simulink model "EV_Bus_Forward_before_readability"  (R2025a)
settings: Solver=ode23t  StartTime=0.0  StopTime=CaseStopTime  MaxStep=Comp.MaxStep  RelTol=1e-5  AbsTol=1e-7
model workspace (MAT data in the model file):
  CaseStopTime = 300
  Comp.Tau = 0.976257419556
  Comp.Limit = 5886
  Comp.InitialForce = 0
  Comp.Enable = 1
  Comp.MinAdaptSpeed = 0.5
  Comp.MeasurementStart = 0
  Comp.MeasurementEnd = 300
  Comp.FilterTau = 0.260335311882
  Comp.Deadband = 44.7421939835
  Comp.ErrorClip = 3531.6
  Comp.MaxRate = 1356.558192
  Comp.LogSampleTime = 0.01
  Comp.MaxStep = 0.01
  MeasuredForceBias = 1114.3044183
  MeasuredTraction = [0 0.01 0.02 0.03 0.04 0.05 0.06 0.07 0.08 0.09 0.1 0.11 ... (60002 elements, 30001x2)]
  P.Mass = 20000
  P.Gravity = 9.81
  P.MotorCount = 2
  P.MotorPower = 400000
  P.MotorPeakTorque = 2500
  P.RegenPeakTorque = 1500
  P.RegenPower = 250000
  P.MaxRPM = 12000
  P.GearRatio = 21
  P.GearEfficiency = 0.97
  P.WheelRadius = 0.5
  P.Cd = 0.65
  P.FrontalArea = 8
  P.Crr = 0.008
  P.AirPressure = 101325
  P.AirGasConstant = 287.05
  P.MotorLag = 0.05
  P.BrakeLag = 0.25
  P.BrakeDelay = 0.1
  P.MaxBrakeTorque = 60000
  P.MaxPressure = 8
  P.DriverKp = 0.22
  P.DriverKi = 0.035
  P.DriverKaw = 2
  P.RegenFadeSpeed = 2
  P.RollingFadeSpeed = 0.2
  P.InitialSpeed = 0
  SignalNames = {'Environment_DesiredSpeed_kmph'; 'Environment_RoadSlope_pct'; 'Environment_AmbientTemp_degC'; 'Driver_Accelerator_pct'; 'Driver_Brake_pct'; 'Powertrain_Controller_MotorCommandTotal_Nm'; 'Powertrain_Controller_BrakeDemandWheel_Nm'; 'Electric_Drive_ActualMotorTotal_Nm'; 'Electric_Drive_ActualMotorEach_Nm'; 'Electric_Drive_ActualMotorSpeed_rpm'; 'Electric_Drive_MechanicalPower_kW'; 'Final_Drive_WheelDriveTorque_Nm'; 'Final_Drive_MotorSpeed_rpm'; 'Final_Drive_FinalDriveRatio'; 'Vehicle_Dynamics_VehicleSpeed_mps'; 'Vehicle_Dynamics_VehicleSpeed_kmph'; 'Vehicle_Dynamics_Acceleration_mps2'; 'Vehicle_Dynamics_AccelerationForce_N'; 'Vehicle_Dynamics_GradientForce_N'; 'Vehicle_Dynamics_RollingResistanceForce_N'; 'Vehicle_Dynamics_AerodynamicForce_N'; 'Vehicle_Dynamics_WheelTractionForce_N'; 'Vehicle_Dynamics_DriveForce_N'; 'Vehicle_Dynamics_FrictionBrakeForce_N'; 'Vehicle_Dynamics_StandstillReaction_N'; 'Vehicle_Dynamics_Distance_m'; 'Pneumatic_Brake_FrictionBrakeTorque_Nm'; 'Pneumatic_Brake_ChamberPressure_bar'; 'MeasuredTraction_N'; 'GenericLossForce_N'; 'CorrectedTraction_N'; 'ResidualError_N'; 'RawDifference_N'; 'AppliedGenericLoss_N'; 'DebiasedMeasuredTraction_N'; 'StationaryForceBias_N'; 'FilteredError_N'; 'AdaptationRate_Nps'}
  SlopeProfile = [0  0; 85  0; 100  4; 140  4; 155  0; 180  -3; 200  0; 300  0]
  SpeedProfile = [0  0; 5  0; 25  40; 55  40; 70  0; 85  0; 105  60; 140  60; 160  40; 180  40; 200  0; 225  0; 245  50; 260  50; 280  0; 300  0]
  TemperatureProfile = [0  25; 150  30; 300  35]
values from neighbouring files (symbols this model uses):
  P =     [EV_Bus_parameters.mat]
(part 1 of 2)
settings Model: Creator=Karuna  LastModifiedBy=Karuna
settings DataIOCC: SignalLogging=off  ReturnWorkspaceOutputs=off

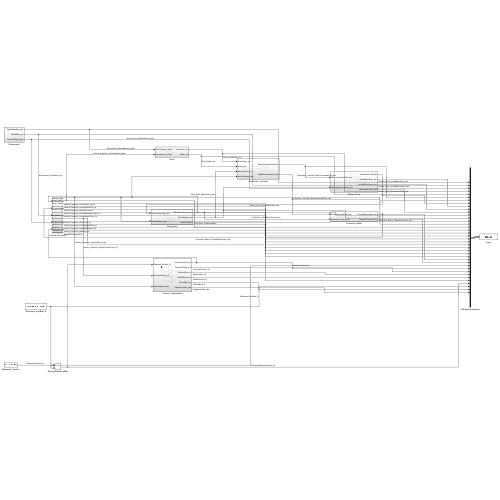
[thumbnail: Simulink's stored preview of the top-level diagram]
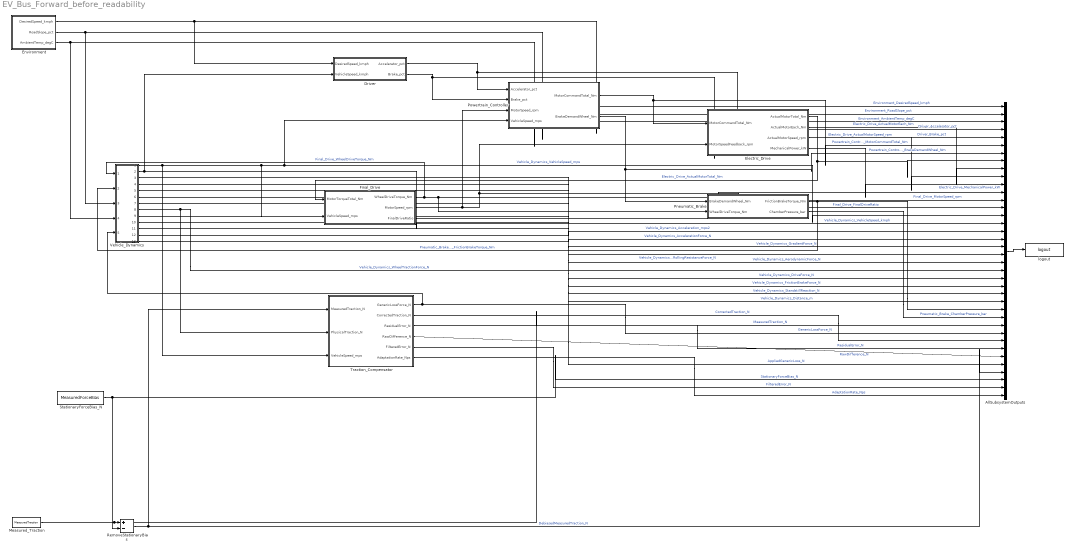
== system EV_Bus_Forward_before_readability ==
  AllSubsystemOutputs : BusCreator  Inputs=38
  Driver : Subsystem  Description=PI speed driver with saturation feedback and integral limits. Non-overlapping accelerator and brake pedals, 0-100%. Minimum 15% holding brake when target <=0.1 km/h.
  Electric_Drive : Subsystem  Description=Equivalent combined model of two identical motors sharing torque equally at common speed. 50 ms torque response; actual torque limited to combined 800 kW drive / 500 kW regen and 5000 / -3000 Nm. Electrical supply assumed available; SOC and thermal dynamics omitted.
  Environment : Subsystem  Description=Linearly interpolated synthetic drive cycle, grade (%) and ambient temperature (degC). Edit SpeedProfile, SlopeProfile and TemperatureProfile in the model workspace.
  Final_Drive : Subsystem  Description=Fixed 21:1 reduction, 0.5 m wheel radius, 97% efficiency. Driving wheel torque = motor torque*21*0.97; regenerative wheel torque = motor torque*21/0.97. RPM comes from actual vehicle speed (no tire slip).
  Measured_Traction : FromWorkspace  Description=MeasuredTraction [relative seconds, signed net traction N], configured by run_EV_Bus_case. Supports arbitrary covered duration and timestamp origin. Original timestamps preserved in logout.sourceTime by the runner.  VariableName=MeasuredTraction
  Pneumatic_Brake : Subsystem  Description=Residual wheel brake demand after actual regenerative torque. Pressure proportional to request, 0.10 s air-line delay and 0.25 s first-order chamber response. 8 bar corresponds to total wheel friction torque 60000 Nm. Reduced-order pneumatic model.
  Powertrain_Controller : Subsystem  Description=Combined command for two equal 400 kW motors. Positive = driving; negative = regeneration. Torque/power envelope, overspeed traction inhibition and regen fade below 2 m/s. Service braking demand is total wheel torque.
  RemoveStationaryBias : Sum  Inputs=+-
  StationaryForceBias_N : Constant  Description=Case-specific measured-force sensor bias. Explicit Bias_N or a user-designated stationary, level, zero-net-traction window; otherwise zero. No universal assumption that the beginning of a recording is stationary.  Value=MeasuredForceBias
  Traction_Compensator : Subsystem  Description=Reusable noise-aware physical loss estimator. All gains, filtering, clipping, bounds and rate limits are in Comp. run_EV_Bus_case imports synchronized measurements/profiles, scales settings from vehicle capability and noise, assesses candidates against a disabled baseline, and checks late-interval performance. Basic Simulink blocks only. Read GENERIC_COMPENSATOR.md for data contract and validity boundaries.
  Vehicle_Dynamics : Subsystem  Description=Physical forward dynamics and traction sum both include AppliedGenericLoss_N. Applied loss = held signed estimate * clamp(v/Comp.MinAdaptSpeed,0,1). Generic motion resistance vanishes at rest; grade is modeled separately. Both force balance identities retained. Ideal standstill constraint can cause abrupt force transitions.
  logout : ToWorkspace  VariableName=logout  SaveFormat=Structure With Time  SampleTime=Comp.LogSampleTime
  wires:
  AllSubsystemOutputs/1 -> logout/1
  Pneumatic_Brake/2(ChamberPressure_bar) -> AllSubsystemOutputs/28  "Pneumatic_Brake_ChamberPressure_bar"
  Final_Drive/3(FinalDriveRatio) -> AllSubsystemOutputs/14  "Final_Drive_FinalDriveRatio"
  Electric_Drive/4(MechanicalPower_kW) -> AllSubsystemOutputs/11  "Electric_Drive_MechanicalPower_kW"
  Electric_Drive/3(ActualMotorSpeed_rpm) -> AllSubsystemOutputs/10  "Electric_Drive_ActualMotorSpeed_rpm"
  Electric_Drive/2(ActualMotorEach_Nm) -> AllSubsystemOutputs/9  "Electric_Drive_ActualMotorEach_Nm"
  Powertrain_Controller/2(BrakeDemandWheel_Nm) -> Pneumatic_Brake/1(BrakeDemandWheel_Nm), AllSubsystemOutputs/7  "Powertrain_Controller_BrakeDemandWheel_Nm"
  Electric_Drive/1(ActualMotorTotal_Nm) -> Final_Drive/1(MotorTorqueTotal_Nm), AllSubsystemOutputs/8  "Electric_Drive_ActualMotorTotal_Nm"
  Powertrain_Controller/1(MotorCommandTotal_Nm) -> Electric_Drive/1(MotorCommandTotal_Nm), AllSubsystemOutputs/6  "Powertrain_Controller_MotorCommandTotal_Nm"
  Final_Drive/2(MotorSpeed_rpm) -> Electric_Drive/2(MotorSpeedFeedback_rpm), AllSubsystemOutputs/13, Powertrain_Controller/3(MotorSpeed_rpm)  "Final_Drive_MotorSpeed_rpm"
  Driver/2(Brake_pct) -> Powertrain_Controller/2(Brake_pct), AllSubsystemOutputs/5  "Driver_Brake_pct"
  Driver/1(Accelerator_pct) -> Powertrain_Controller/1(Accelerator_pct), AllSubsystemOutputs/4  "Driver_Accelerator_pct"
  Environment/1(DesiredSpeed_kmph) -> Driver/1(DesiredSpeed_kmph), AllSubsystemOutputs/1  "Environment_DesiredSpeed_kmph"
  StationaryForceBias_N/1 -> AllSubsystemOutputs/36, RemoveStationaryBias/2  "StationaryForceBias_N"
  Measured_Traction/1 -> RemoveStationaryBias/1, AllSubsystemOutputs/29  "MeasuredTraction_N"
  Vehicle_Dynamics/12(Distance_m) -> AllSubsystemOutputs/26  "Vehicle_Dynamics_Distance_m"
  Vehicle_Dynamics/11(StandstillReaction_N) -> AllSubsystemOutputs/25  "Vehicle_Dynamics_StandstillReaction_N"
  Vehicle_Dynamics/10(FrictionBrakeForce_N) -> AllSubsystemOutputs/24  "Vehicle_Dynamics_FrictionBrakeForce_N"
  Vehicle_Dynamics/9(DriveForce_N) -> AllSubsystemOutputs/23  "Vehicle_Dynamics_DriveForce_N"
  Vehicle_Dynamics/7(AerodynamicForce_N) -> AllSubsystemOutputs/21  "Vehicle_Dynamics_AerodynamicForce_N"
  Vehicle_Dynamics/6(RollingResistanceForce_N) -> AllSubsystemOutputs/20  "Vehicle_Dynamics_RollingResistanceForce_N"
  Vehicle_Dynamics/5(GradientForce_N) -> AllSubsystemOutputs/19  "Vehicle_Dynamics_GradientForce_N"
  Vehicle_Dynamics/4(AccelerationForce_N) -> AllSubsystemOutputs/18  "Vehicle_Dynamics_AccelerationForce_N"
  Vehicle_Dynamics/3(Acceleration_mps2) -> AllSubsystemOutputs/17  "Vehicle_Dynamics_Acceleration_mps2"
  Environment/3(AmbientTemp_degC) -> AllSubsystemOutputs/3, Vehicle_Dynamics/4(AmbientTemp_degC)  "Environment_AmbientTemp_degC"
  Environment/2(RoadSlope_pct) -> Vehicle_Dynamics/3(RoadSlope_pct), AllSubsystemOutputs/2  "Environment_RoadSlope_pct"
  Pneumatic_Brake/1(FrictionBrakeTorque_Nm) -> Vehicle_Dynamics/2(FrictionBrakeTorque_Nm), AllSubsystemOutputs/27  "Pneumatic_Brake_FrictionBrakeTorque_Nm"
  Final_Drive/1(WheelDriveTorque_Nm) -> Pneumatic_Brake/2(WheelDriveTorque_Nm), AllSubsystemOutputs/12, Vehicle_Dynamics/1(WheelDriveTorque_Nm)  "Final_Drive_WheelDriveTorque_Nm"
  Vehicle_Dynamics/2(VehicleSpeed_kmph) -> Driver/2(VehicleSpeed_kmph), AllSubsystemOutputs/16  "Vehicle_Dynamics_VehicleSpeed_kmph"
  Vehicle_Dynamics/13(AppliedGenericLoss_N) -> AllSubsystemOutputs/34  "AppliedGenericLoss_N"
  Traction_Compensator/6(AdaptationRate_Nps) -> AllSubsystemOutputs/38  "AdaptationRate_Nps"
  Traction_Compensator/5(FilteredError_N) -> AllSubsystemOutputs/37  "FilteredError_N"
  RemoveStationaryBias/1 -> AllSubsystemOutputs/35, Traction_Compensator/1(MeasuredTraction_N)  "DebiasedMeasuredTraction_N"
  Vehicle_Dynamics/8(WheelTractionForce_N) -> Traction_Compensator/2(PhysicalTraction_N), AllSubsystemOutputs/22  "Vehicle_Dynamics_WheelTractionForce_N"
  Traction_Compensator/1(GenericLossForce_N) -> AllSubsystemOutputs/30, Vehicle_Dynamics/5(GenericLossForce_N)  "GenericLossForce_N"
  Traction_Compensator/2(CorrectedTraction_N) -> AllSubsystemOutputs/31  "CorrectedTraction_N"
  Traction_Compensator/3(ResidualError_N) -> AllSubsystemOutputs/32  "ResidualError_N"
  Traction_Compensator/4(RawDifference_N) -> AllSubsystemOutputs/33  "RawDifference_N"
  Vehicle_Dynamics/1(VehicleSpeed_mps) -> Powertrain_Controller/4(VehicleSpeed_mps), AllSubsystemOutputs/15, Final_Drive/2(VehicleSpeed_mps), Traction_Compensator/3(VehicleSpeed_mps)  "Vehicle_Dynamics_VehicleSpeed_mps"
